simulink model "ATOM_parking_chain"  (R2026a)
settings: Solver=ode4  StopTime=100  FixedStep=0.01
StopFcn:
  | % Put every new figure in the same MATLAB Figures window as a docked tab.
  | set(groot, 'defaultFigureWindowStyle', 'docked');
  | 
  | if exist('costmap_active', 'var') && ...
  |         exist('vehicle', 'var') && ...
  |         exist('parking_path', 'var') && ...
  |         ~isempty(parking_path)
  | 
  |     plotPlan(costmap_active, vehicle, parking_path);
  | 
  | else
  | 
  |     warning('No valid parking path is available for plotting.');
  | 
  | end
  | 
  | PlotControllerReferences( ...
  |     out.controller_reference_log);
  | 
  | PlotControllerTracking( ...
  |     out.controller_tracking_log);
undefined symbols (not defined in the file): lateral, longitudinal, stanley, vehicle
(part 1 of 11)
settings Model: Creator=husain5  LastModifiedBy=husain5
settings HardwareCC: ProdBitPerLong=64.0  ProdHWDeviceType=Intel->x86-64 (Linux 64)

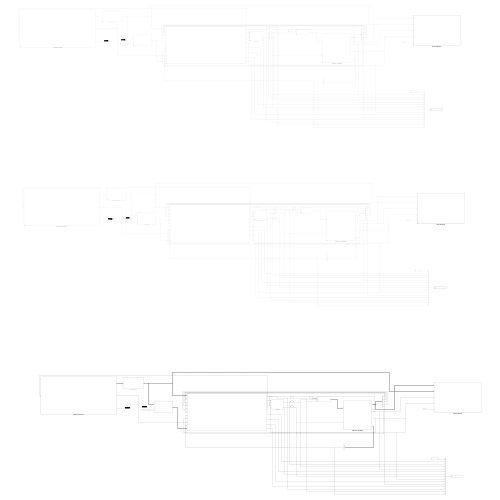
[thumbnail: Simulink's stored preview of the top-level diagram]
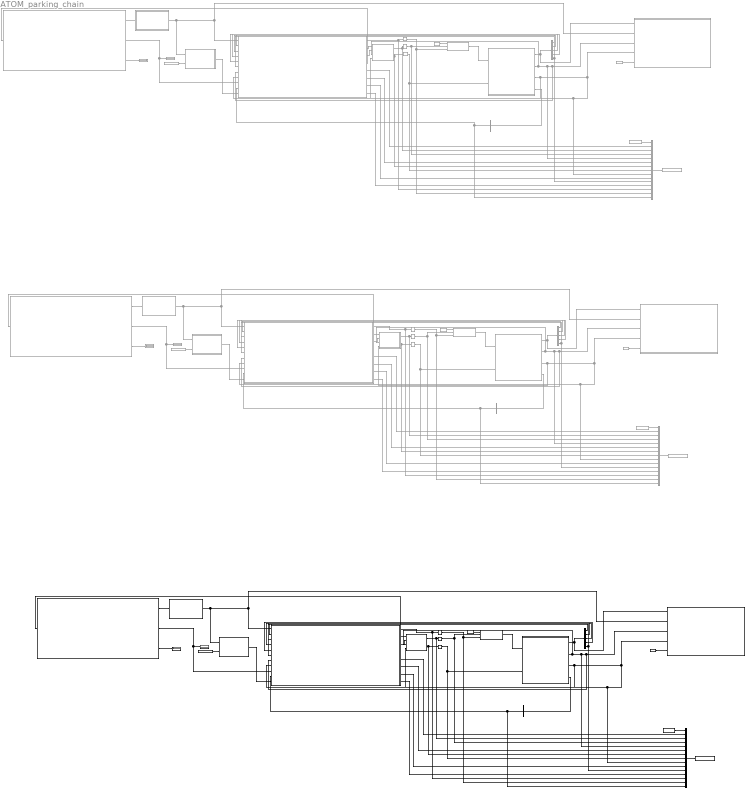
== system ATOM_parking_chain ==
  Bus Assignment : BusAssignment  Commented=on  AssignedSignals=lateral.steering_tire_angle,longitudinal.acceleration
  Bus Assignment1 : BusAssignment  Commented=on  AssignedSignals=lateral.steering_tire_angle,longitudinal.acceleration
  Bus Assignment2 : BusAssignment  AssignedSignals=lateral.steering_tire_angle,longitudinal.acceleration
  Bus Selector1 : BusSelector  Commented=on  OutputSignals=pose.position.x,pose.position.y,pose.orientation.z,pose.orientation.w,twist.linear.x
  Bus Selector2 : BusSelector  Commented=on  OutputSignals=pose.position.x,pose.position.y,pose.orientation.z,pose.orientation.w,twist.linear.x
  Bus Selector3 : BusSelector  Commented=on  OutputSignals=acceleration.linear.x
  Bus Selector4 : BusSelector  Commented=on  OutputSignals=acceleration.linear.x
  Bus Selector5 : BusSelector  OutputSignals=pose.position.x,pose.position.y,pose.orientation.z,pose.orientation.w,twist.linear.x
  Bus Selector6 : BusSelector  OutputSignals=acceleration.linear.x
  Constant : Constant  Commented=on  Value=0  OutDataTypeStr=Bus: ControlCMDBus
  Constant1 : Constant  Commented=on  Value=vehicle.sim.steer_rate_lim
  Constant2 : Constant  Commented=on  Value=0  OutDataTypeStr=Bus: ControlCMDBus
  Constant3 : Constant  Commented=on  Value=vehicle.sim.steer_rate_lim
  Constant4 : Constant  Value=0  OutDataTypeStr=Bus: ControlCMDBus
  Constant5 : Constant  Value=vehicle.sim.steer_rate_lim
  Digital Clock : DigitalClock  Commented=on  SampleTime=0.04
  Digital Clock1 : DigitalClock  Commented=on  SampleTime=0.04
  Digital Clock2 : DigitalClock  SampleTime=0.04
  Display{,1..3} (4 alike) : Display  Commented=on
  Display4 : Display
  Display5 : Display
  From Workspace1 : FromWorkspace  Commented=on  VariableName=veh
  From Workspace2 : FromWorkspace  Commented=on  VariableName=veh
  From Workspace3 : FromWorkspace  VariableName=veh
  Mux1 : Mux  Commented=on  Inputs=15
  Mux2 : Mux  Commented=on  Inputs=15
  Mux3 : Mux  Inputs=15
  Parking Scenario : Subsystem  Commented=on
  Parking Scenario1 : Subsystem  Commented=on
  Parking Scenario2 : Subsystem
  Plot vehicle1 : Subsystem  Commented=on
  Plot vehicle2 : Subsystem  Commented=on
  Plot vehicle3 : Subsystem
  Subsystem : Subsystem  Commented=on
  Subsystem1 : Subsystem  Commented=on
  Subsystem2 : Subsystem
  To Workspace1 : ToWorkspace  Commented=on  VariableName=controller_tracking_log  SaveFormat=Timeseries  SampleTime=-1
  To Workspace2 : ToWorkspace  Commented=on  VariableName=controller_tracking_log2  SaveFormat=Timeseries  SampleTime=-1
  To Workspace3 : ToWorkspace  VariableName=controller_tracking_log  SaveFormat=Timeseries  SampleTime=-1
  Transport Delay : TransportDelay  Commented=on  DelayTime=vehicle.sim.acc_time_delay
  Transport Delay{1..2,4..5} (4 alike) : TransportDelay  Commented=on  DelayTime=vehicle.sim.steer_time_delay
  Transport Delay3 : TransportDelay  Commented=on  DelayTime=vehicle.sim.acc_time_delay
  Transport Delay6 : TransportDelay  DelayTime=vehicle.sim.acc_time_delay
  Transport Delay7 : TransportDelay  DelayTime=vehicle.sim.steer_time_delay
  Transport Delay8 : TransportDelay  DelayTime=vehicle.sim.steer_time_delay
  Vehicle_Model : Subsystem  Commented=on
  Vehicle_Model1 : Subsystem  Commented=on
  Vehicle_Model2 : Subsystem
  parking_velocity_smoother : Subsystem  Commented=on
  parking_velocity_smoother1 : Subsystem  Commented=on
  parking_velocity_smoother2 : Subsystem
  steeringRatetoAngle : Subsystem  Commented=on
  steeringRatetoAngle1 : Subsystem  Commented=on
  steeringRatetoAngle2 : Subsystem
  time_parameterization : Subsystem  Commented=on
  time_parameterization1 : Subsystem  Commented=on
  time_parameterization2 : Subsystem
  wires:
  From Workspace2/1 -> Plot vehicle1/5(veh)
  Constant/1 -> Bus Assignment/1
  Subsystem/4(segment_done) -> Parking Scenario/1(segment_done)
  Subsystem/5(df_ref_out) -> Mux1/2
  Subsystem/1("a_cmd ") -> Transport Delay/1, Mux1/13
  Parking Scenario/1(traj) -> parking_velocity_smoother/1(trajectory_in)
  Bus Selector2/3 -> Subsystem/4(qz)  "<z>"
  Bus Selector2/5 -> Mux1/11, Subsystem/6(vx)  "<x>"
  Bus Selector2/1 -> Subsystem/2(X)  "<x>"
  parking_velocity_smoother/1(trajectory_out) -> time_parameterization/1(trajectory_in), Subsystem/1(planning/scenario_planning/scenario_selector/trajectory), Plot vehicle1/2(planning/scenario_planning/scenario_selector/trajectory)
  Mux1/1 -> To Workspace1/1
  Bus Selector2/4 -> Subsystem/5(qw)  "<w>"
  Subsystem/7(v_ref_out) -> Mux1/10
  Transport Delay1/1 -> Mux1/4, Bus Assignment/2
  Vehicle_Model/3(steer_rear) -> steeringRatetoAngle/4(dr_measured), Mux1/9, Subsystem/8(dr), Plot vehicle1/4(steer_rear)
  Digital Clock/1 -> Mux1/1
  Bus Assignment/1 -> Vehicle_Model/1(command)
  Transport Delay/1 -> Mux1/14, Bus Assignment/3
  Parking Scenario/2(active_segment) -> Subsystem/9(active_segment), Display/1
  Vehicle_Model/1(kinematic) -> Plot vehicle1/1(localization/kinematic_state), Bus Selector2/1  "/localization/kinematic_state"
  Bus Selector3/1 -> Mux1/15, Subsystem/10(ax_meas)  "<x>"
  Transport Delay2/1 -> Mux1/8, Vehicle_Model/2(rear_steer_commanf)
  Bus Selector2/2 -> Subsystem/3(Y)  "<y>"
  Vehicle_Model/2(steer_front) -> steeringRatetoAngle/3(df_measured), Mux1/5, Subsystem/7(df), Plot vehicle1/3(steer_front)
  Parking Scenario/3(maneuver_complete) -> Display1/1
  Subsystem/6(dr_ref_out) -> Mux1/6
  Subsystem/8(a_ref_out) -> Mux1/12
  Vehicle_Model/4(accel) -> Bus Selector3/1  "/localization/acceleration"
  time_parameterization/1(reference_out) -> Subsystem/11(reference_out)
  Constant1/1 -> time_parameterization/2(steer_rate_limit)
  steeringRatetoAngle/2(dr_angle_cmd) -> Transport Delay2/1, Mux1/7
  steeringRatetoAngle/1(df_angle_cmd) -> Transport Delay1/1, Mux1/3
  Subsystem/2(df_cmd) -> steeringRatetoAngle/1(df_rate_cmd)
  Subsystem/3(dr_cmd) -> steeringRatetoAngle/2(dr_rate_cmd)
  Vehicle_Model1/4(accel) -> Bus Selector4/1  "/localization/acceleration"
  Vehicle_Model1/3(steer_rear) -> steeringRatetoAngle1/4(dr_measured), Mux2/9, Subsystem1/8(dr), Plot vehicle2/4(steer_rear)
  Subsystem1/1("a_cmd ") -> Transport Delay3/1, Mux2/13
  Bus Selector1/5 -> Mux2/11, Subsystem1/6(vx)  "<x>"
  Transport Delay4/1 -> Bus Assignment1/2, Mux2/4
  Bus Selector4/1 -> Subsystem1/10(ax_meas), Mux2/15  "<x>"
  Transport Delay5/1 -> Vehicle_Model1/2(rear_steer_commanf), Mux2/8
  Mux2/1 -> To Workspace2/1
  Constant2/1 -> Bus Assignment1/1
  parking_velocity_smoother1/1(trajectory_out) -> time_parameterization1/1(trajectory_in), Subsystem1/1(planning/scenario_planning/scenario_selector/trajectory), Plot vehicle2/2(planning/scenario_planning/scenario_selector/trajectory)
  Subsystem1/6(dr_ref_out) -> Mux2/6
  Parking Scenario1/2(active_segment) -> Subsystem1/9(active_segment), Display2/1
  Subsystem1/5(df_ref_out) -> Mux2/2
  Subsystem1/2(df_cmd) -> steeringRatetoAngle1/1(df_rate_cmd)
  Subsystem1/8(a_ref_out) -> Mux2/12
  time_parameterization1/1(reference_out) -> Subsystem1/11(reference_out)
  Transport Delay3/1 -> Mux2/14, Bus Assignment1/3
  Parking Scenario1/1(traj) -> parking_velocity_smoother1/1(trajectory_in)
  Bus Selector1/2 -> Subsystem1/3(Y)  "<y>"
  Vehicle_Model1/2(steer_front) -> steeringRatetoAngle1/3(df_measured), Mux2/5, Subsystem1/7(df), Plot vehicle2/3(steer_front)
  Constant3/1 -> time_parameterization1/2(steer_rate_limit)
  From Workspace1/1 -> Plot vehicle2/5(veh)
  steeringRatetoAngle1/2(dr_angle_cmd) -> Transport Delay5/1, Mux2/7
  Subsystem1/7(v_ref_out) -> Mux2/10
  Digital Clock1/1 -> Mux2/1
  Subsystem1/3(dr_cmd) -> steeringRatetoAngle1/2(dr_rate_cmd)
  Bus Assignment1/1 -> Vehicle_Model1/1(command)
  Parking Scenario1/3(maneuver_complete) -> Display3/1
  Vehicle_Model1/1(kinematic) -> Plot vehicle2/1(localization/kinematic_state), Bus Selector1/1  "/localization/kinematic_state"
  steeringRatetoAngle1/1(df_angle_cmd) -> Mux2/3, Transport Delay4/1
  Bus Selector1/3 -> Subsystem1/4(qz)  "<z>"
  Bus Selector1/4 -> Subsystem1/5(qw)  "<w>"
  Bus Selector1/1 -> Subsystem1/2(X)  "<x>"
  Subsystem1/4(segment_done) -> Parking Scenario1/1(segment_done)
  Bus Selector5/3 -> Subsystem2/4(qz)  "<z>"
  Parking Scenario2/3(maneuver_complete) -> Display5/1
  parking_velocity_smoother2/1(trajectory_out) -> time_parameterization2/1(trajectory_in), Subsystem2/1(planning/scenario_planning/scenario_selector/trajectory), Plot vehicle3/2(planning/scenario_planning/scenario_selector/trajectory)
  Bus Selector5/2 -> Subsystem2/3(Y)  "<y>"
  Subsystem2/1("a_cmd ") -> Transport Delay6/1, Mux3/13
  Bus Selector6/1 -> Subsystem2/10(ax_meas), Mux3/15  "<x>"
  Vehicle_Model2/4(accel) -> Bus Selector6/1  "/localization/acceleration"
  Subsystem2/8(a_ref_out) -> Mux3/12
  Vehicle_Model2/2(steer_front) -> steeringRatetoAngle2/3(df_measured), Mux3/5, Subsystem2/7(df), Plot vehicle3/3(steer_front)
  Subsystem2/6(dr_ref_out) -> Mux3/6
  Bus Selector5/1 -> Subsystem2/2(X)  "<x>"
  time_parameterization2/1(reference_out) -> Subsystem2/11(reference_out)
  Subsystem2/7(v_ref_out) -> Mux3/10
  Constant5/1 -> time_parameterization2/2(steer_rate_limit)
  Vehicle_Model2/3(steer_rear) -> steeringRatetoAngle2/4(dr_measured), Mux3/9, Subsystem2/8(dr), Plot vehicle3/4(steer_rear)
  Subsystem2/4(segment_done) -> Parking Scenario2/1(segment_done)
  Constant4/1 -> Bus Assignment2/1
  steeringRatetoAngle2/2(dr_angle_cmd) -> Transport Delay8/1, Mux3/7
  Subsystem2/2(df_cmd) -> steeringRatetoAngle2/1(df_rate_cmd)
  Digital Clock2/1 -> Mux3/1
  Transport Delay6/1 -> Mux3/14, Bus Assignment2/3
  Mux3/1 -> To Workspace3/1
  Parking Scenario2/1(traj) -> parking_velocity_smoother2/1(trajectory_in)
  Bus Selector5/4 -> Subsystem2/5(qw)  "<w>"
  Subsystem2/5(df_ref_out) -> Mux3/2
  Bus Selector5/5 -> Mux3/11, Subsystem2/6(vx)  "<x>"
  steeringRatetoAngle2/1(df_angle_cmd) -> Mux3/3, Transport Delay7/1
  Transport Delay7/1 -> Bus Assignment2/2, Mux3/4
  Transport Delay8/1 -> Vehicle_Model2/2(rear_steer_commanf), Mux3/8
  Vehicle_Model2/1(kinematic) -> Plot vehicle3/1(localization/kinematic_state), Bus Selector5/1  "/localization/kinematic_state"
  Bus Assignment2/1 -> Vehicle_Model2/1(command)
  Parking Scenario2/2(active_segment) -> Subsystem2/9(active_segment), Display4/1
  From Workspace3/1 -> Plot vehicle3/5(veh)
  Subsystem2/3(dr_cmd) -> steeringRatetoAngle2/2(dr_rate_cmd)

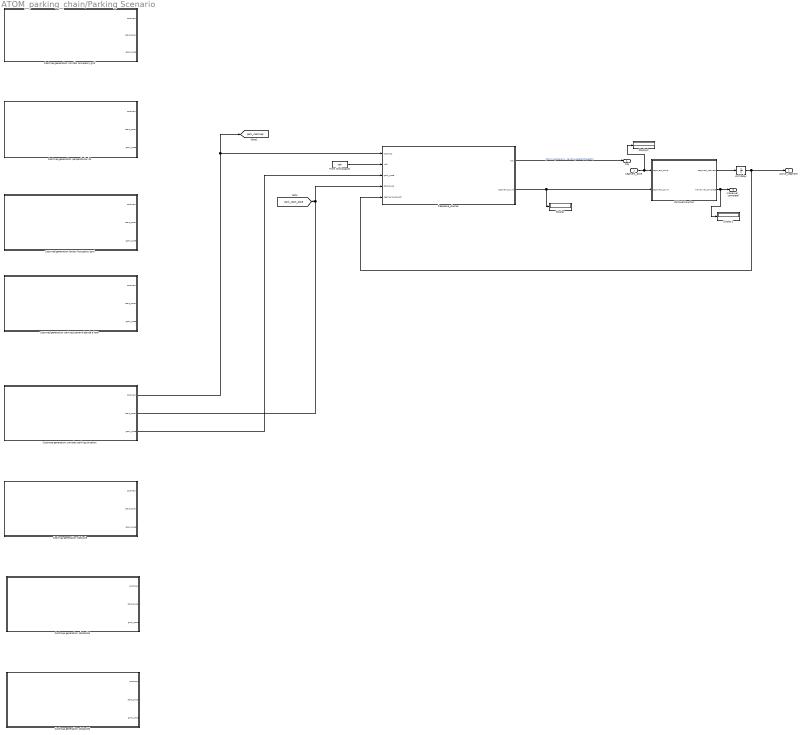
== system ATOM_parking_chain/Parking Scenario ==
  segment_done : Inport
  Costmap generation: complex parking situation : Subsystem
  Costmap generation: corridor occupancy grid : Subsystem
  Costmap generation: empty occupancy grid : Subsystem
  Costmap generation: obstacle : Subsystem
  Costmap generation: obstacle1 : Subsystem
  Costmap generation: obstacle2 : Subsystem
  Costmap generation: parking scenario beside a lane : Subsystem
  Costmap generation: perpendicular lot : Subsystem
  Display : Display
  Display1 : Display
  Display2 : Display
  From Workspace1 : FromWorkspace  VariableName=veh
  MATLAB Function : MATLAB Function  TreatAsAtomicUnit=on
  Unit Delay : UnitDelay  InitialCondition=1  SampleTime=0.04
  freespace_planner : Subsystem
  traj : Outport
  active_segment : Outport  Port=2
  maneuver_complete : Outport  Port=3
  tag scope: park_costmap=global, park_start_pose=global
  wires:
  Costmap generation: complex parking situation/1(costmap) -> [park_costmap], freespace_planner/1(costmap)
  From Workspace1/1 -> freespace_planner/2(veh)
  Costmap generation: complex parking situation/3(goal_pose) -> freespace_planner/3(goal_pose)
  Costmap generation: complex parking situation/2(start_pose) -> freespace_planner/4(start_pose), [park_start_pose]
  freespace_planner/1(traj) -> traj/1  "/planning/scenario_planning/scenario_selector/trajectory"
  Unit Delay/1 -> freespace_planner/5(segment_request), active_segment/1
  freespace_planner/2(segment_count) -> Display/1, MATLAB Function/2(segment_count)
  segment_done/1 -> Display2/1, MATLAB Function/1(segment_done)
  MATLAB Function/1(segment_request) -> Unit Delay/1
  MATLAB Function/2(maneuver_complete) -> Display1/1, maneuver_complete/1

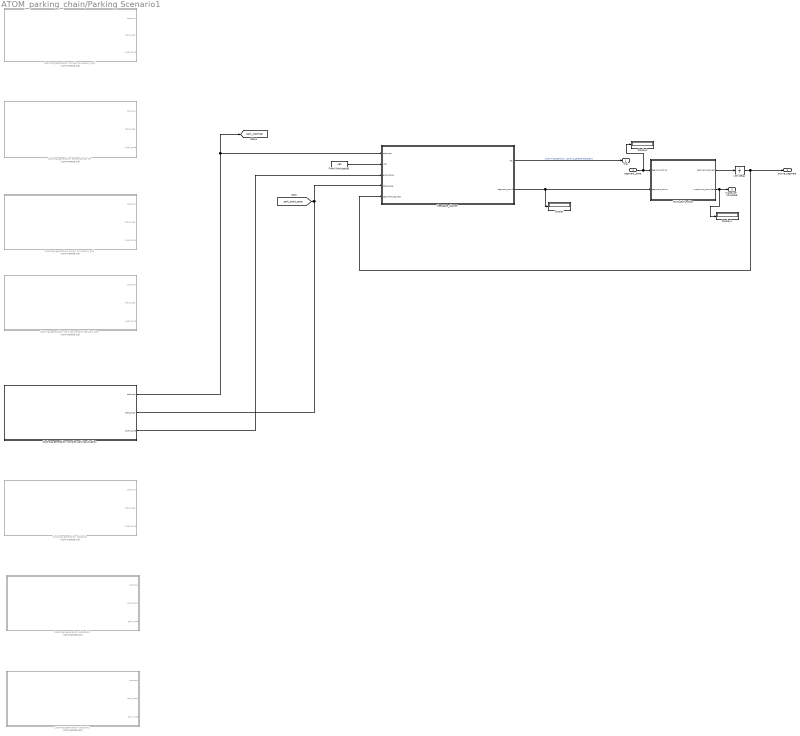
== system ATOM_parking_chain/Parking Scenario1 ==
  segment_done : Inport
  Costmap generation: complex parking situation : Subsystem
  Costmap generation: corridor occupancy grid : Subsystem  Commented=on
  Costmap generation: empty occupancy grid : Subsystem  Commented=on
  Costmap generation: obstacle : Subsystem  Commented=on
  Costmap generation: obstacle1 : Subsystem  Commented=on
  Costmap generation: obstacle2 : Subsystem  Commented=on
  Costmap generation: parking scenario beside a lane : Subsystem  Commented=on
  Costmap generation: perpendicular lot : Subsystem  Commented=on
  Display : Display
  Display1 : Display
  Display2 : Display
  From Workspace1 : FromWorkspace  VariableName=veh
  MATLAB Function : MATLAB Function  TreatAsAtomicUnit=on
  Unit Delay : UnitDelay  InitialCondition=1  SampleTime=0.04
  freespace_planner : Subsystem
  traj : Outport
  active_segment : Outport  Port=2
  maneuver_complete : Outport  Port=3
  tag scope: park_costmap=global, park_start_pose=global
  wires:
  Costmap generation: complex parking situation/1(costmap) -> [park_costmap], freespace_planner/1(costmap)
  From Workspace1/1 -> freespace_planner/2(veh)
  Costmap generation: complex parking situation/3(goal_pose) -> freespace_planner/3(goal_pose)
  Costmap generation: complex parking situation/2(start_pose) -> freespace_planner/4(start_pose), [park_start_pose]
  freespace_planner/1(traj) -> traj/1  "/planning/scenario_planning/scenario_selector/trajectory"
  Unit Delay/1 -> freespace_planner/5(segment_request), active_segment/1
  freespace_planner/2(segment_count) -> Display/1, MATLAB Function/2(segment_count)
  segment_done/1 -> Display2/1, MATLAB Function/1(segment_done)
  MATLAB Function/1(segment_request) -> Unit Delay/1
  MATLAB Function/2(maneuver_complete) -> Display1/1, maneuver_complete/1

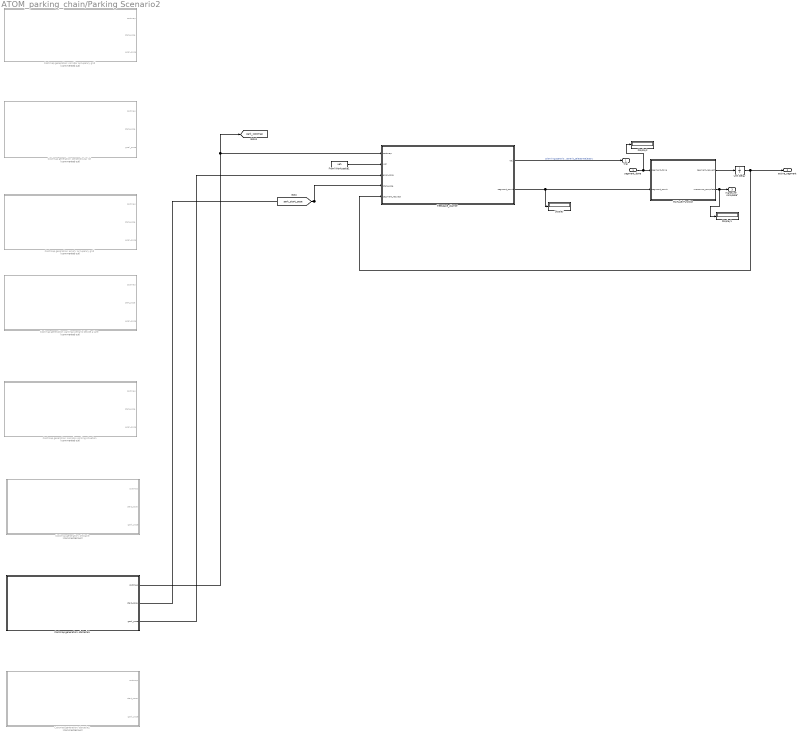
== system ATOM_parking_chain/Parking Scenario2 ==
  segment_done : Inport
  Costmap generation: complex parking situation : Subsystem  Commented=on
  Costmap generation: corridor occupancy grid : Subsystem  Commented=on
  Costmap generation: empty occupancy grid : Subsystem  Commented=on
  Costmap generation: obstacle : Subsystem  Commented=on
  Costmap generation: obstacle1 : Subsystem
  Costmap generation: obstacle2 : Subsystem  Commented=on
  Costmap generation: parking scenario beside a lane : Subsystem  Commented=on
  Costmap generation: perpendicular lot : Subsystem  Commented=on
  Display : Display
  Display1 : Display
  Display2 : Display
  From Workspace1 : FromWorkspace  VariableName=veh
  MATLAB Function : MATLAB Function  TreatAsAtomicUnit=on
  Unit Delay : UnitDelay  InitialCondition=1  SampleTime=0.04
  freespace_planner : Subsystem
  traj : Outport
  active_segment : Outport  Port=2
  maneuver_complete : Outport  Port=3
  tag scope: park_costmap=global, park_start_pose=global
  wires:
  Costmap generation: obstacle1/1(costmap) -> [park_costmap], freespace_planner/1(costmap)
  From Workspace1/1 -> freespace_planner/2(veh)
  Costmap generation: obstacle1/3(goal_pose) -> freespace_planner/3(goal_pose)
  Costmap generation: obstacle1/2(start_pose) -> freespace_planner/4(start_pose), [park_start_pose]
  freespace_planner/1(traj) -> traj/1  "/planning/scenario_planning/scenario_selector/trajectory"
  Unit Delay/1 -> freespace_planner/5(segment_request), active_segment/1
  freespace_planner/2(segment_count) -> Display/1, MATLAB Function/2(segment_count)
  segment_done/1 -> Display2/1, MATLAB Function/1(segment_done)
  MATLAB Function/1(segment_request) -> Unit Delay/1
  MATLAB Function/2(maneuver_complete) -> Display1/1, maneuver_complete/1

== system ATOM_parking_chain/Plot vehicle1 ==
  localization/kinematic_state : Inport
  planning/scenario_planning/scenario_selector/trajectory : Inport  Port=2
  steer_front : Inport  Port=3
  steer_rear : Inport  Port=4
  veh : Inport  Port=5
  Constant : Constant  Value=vehicle.param.wheel_base
  Plot Vehicle Rear reference frame : MATLAB Function  TreatAsAtomicUnit=on
  Plot vehicle Front reference frame : MATLAB Function  TreatAsAtomicUnit=on
  RearToFrontOdometry : MATLAB Function  TreatAsAtomicUnit=on
  SetStanleyTrajectory : Subsystem
  wires:
  steer_rear/1 -> Plot vehicle Front reference frame/3(steer_rear), Plot Vehicle Rear reference frame/3(steer_rear)
  veh/1 -> Plot vehicle Front reference frame/4(veh), Plot Vehicle Rear reference frame/4(veh)
  steer_front/1 -> Plot Vehicle Rear reference frame/2(steer_front), Plot vehicle Front reference frame/2(steer_front)
  Constant/1 -> RearToFrontOdometry/2(wheel_base)
  localization/kinematic_state/1 -> Plot Vehicle Rear reference frame/1(kinematic), RearToFrontOdometry/1(rear_pose)
  planning/scenario_planning/scenario_selector/trajectory/1 -> SetStanleyTrajectory/1(ref_traj), Plot Vehicle Rear reference frame/5(traj)
  RearToFrontOdometry/1(front_pose) -> SetStanleyTrajectory/2(ego_pose), Plot vehicle Front reference frame/1(kinematic)
  SetStanleyTrajectory/1(trajectory_out) -> Plot vehicle Front reference frame/5(traj)
  [park_costmap] -> Plot Vehicle Rear reference frame/6(costmap)

== system ATOM_parking_chain/Plot vehicle2 ==
  localization/kinematic_state : Inport
  planning/scenario_planning/scenario_selector/trajectory : Inport  Port=2
  steer_front : Inport  Port=3
  steer_rear : Inport  Port=4
  veh : Inport  Port=5
  Constant : Constant  Value=vehicle.param.wheel_base
  Plot Vehicle Rear reference frame : MATLAB Function  TreatAsAtomicUnit=on
  Plot vehicle Front reference frame : MATLAB Function  TreatAsAtomicUnit=on
  RearToFrontOdometry : MATLAB Function  TreatAsAtomicUnit=on
  SetStanleyTrajectory : Subsystem
  wires:
  steer_rear/1 -> Plot vehicle Front reference frame/3(steer_rear), Plot Vehicle Rear reference frame/3(steer_rear)
  veh/1 -> Plot vehicle Front reference frame/4(veh), Plot Vehicle Rear reference frame/4(veh)
  steer_front/1 -> Plot Vehicle Rear reference frame/2(steer_front), Plot vehicle Front reference frame/2(steer_front)
  Constant/1 -> RearToFrontOdometry/2(wheel_base)
  localization/kinematic_state/1 -> Plot Vehicle Rear reference frame/1(kinematic), RearToFrontOdometry/1(rear_pose)
  planning/scenario_planning/scenario_selector/trajectory/1 -> SetStanleyTrajectory/1(ref_traj), Plot Vehicle Rear reference frame/5(traj)
  RearToFrontOdometry/1(front_pose) -> SetStanleyTrajectory/2(ego_pose), Plot vehicle Front reference frame/1(kinematic)
  SetStanleyTrajectory/1(trajectory_out) -> Plot vehicle Front reference frame/5(traj)
  [park_costmap] -> Plot Vehicle Rear reference frame/6(costmap)

== system ATOM_parking_chain/Plot vehicle3 ==
  localization/kinematic_state : Inport
  planning/scenario_planning/scenario_selector/trajectory : Inport  Port=2
  steer_front : Inport  Port=3
  steer_rear : Inport  Port=4
  veh : Inport  Port=5
  Constant : Constant  Value=vehicle.param.wheel_base
  Plot Vehicle Rear reference frame : MATLAB Function  TreatAsAtomicUnit=on
  Plot vehicle Front reference frame : MATLAB Function  TreatAsAtomicUnit=on
  RearToFrontOdometry : MATLAB Function  TreatAsAtomicUnit=on
  SetStanleyTrajectory : Subsystem
  wires:
  steer_rear/1 -> Plot vehicle Front reference frame/3(steer_rear), Plot Vehicle Rear reference frame/3(steer_rear)
  veh/1 -> Plot vehicle Front reference frame/4(veh), Plot Vehicle Rear reference frame/4(veh)
  steer_front/1 -> Plot Vehicle Rear reference frame/2(steer_front), Plot vehicle Front reference frame/2(steer_front)
  Constant/1 -> RearToFrontOdometry/2(wheel_base)
  localization/kinematic_state/1 -> Plot Vehicle Rear reference frame/1(kinematic), RearToFrontOdometry/1(rear_pose)
  planning/scenario_planning/scenario_selector/trajectory/1 -> SetStanleyTrajectory/1(ref_traj), Plot Vehicle Rear reference frame/5(traj)
  RearToFrontOdometry/1(front_pose) -> SetStanleyTrajectory/2(ego_pose), Plot vehicle Front reference frame/1(kinematic)
  SetStanleyTrajectory/1(trajectory_out) -> Plot vehicle Front reference frame/5(traj)
  [park_costmap] -> Plot Vehicle Rear reference frame/6(costmap)

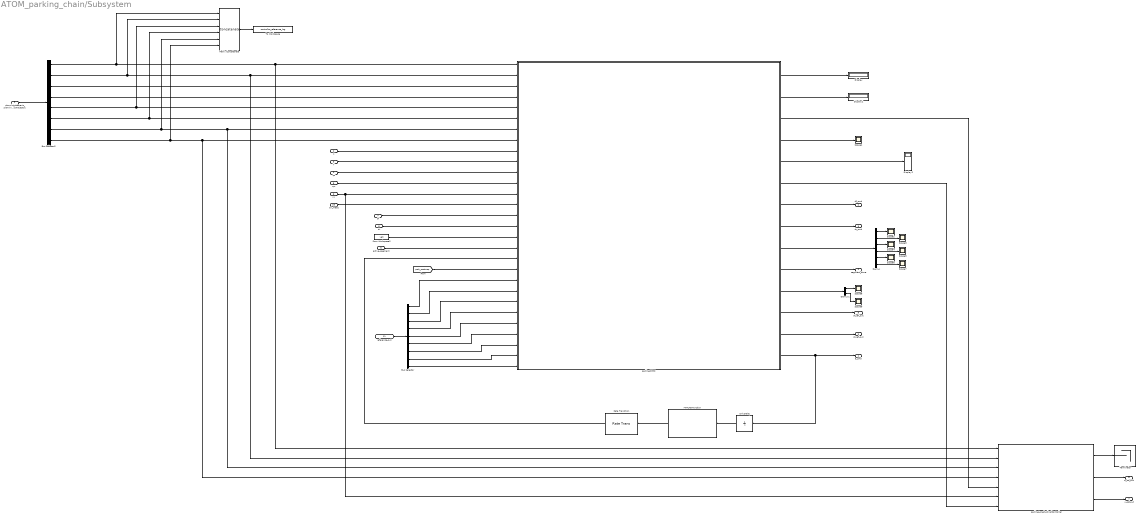
== system ATOM_parking_chain/Subsystem ==
  planning/scenario_planning/scenario_selector/trajectory : Inport
  X : Inport  Port=2
  Y : Inport  Port=3
  qz : Inport  Port=4
  qw : Inport  Port=5
  vx : Inport  Port=6
  df : Inport  Port=7
  dr : Inport  Port=8
  active_segment : Inport  Port=9
  ax_meas : Inport  Port=10
  reference_out : Inport  Port=11  OutDataTypeStr=Bus: ParkingReferenceBus  PortDimensions=1
  Bus Selector : BusSelector  OutputSignals=t_ref,s_ref,x_ref,y_ref,psi_ref,v_ref,a_ref,df_nom,dr_nom
  Bus Selector2 : BusSelector  OutputSignals=pose.position.x,pose.position.y,pose.orientation.qz,pose.orientation.qw,front_wheel_angle_rad,rear_wheel_angle_rad,longitudinal_velocity_mps,acceleration_mps2
  Demux : Demux  Outputs=6
  Demux1 : Demux  Outputs=2
  Display : Display
  Display1 : Display
  Display2 : Display
  From Workspace2 : FromWorkspace  VariableName=veh
  MATLAB Function : MATLAB Function  TreatAsAtomicUnit=on
  Matrix Concatenate : Concatenate  NumInputs=6  Mode=Multidimensional array  ConcatenateDimension=2
  Rate Transition : RateTransition  OutPortSampleTime=0.04
  Scope{1..9} (9 alike) : Scope
      Scope1 settings: ActiveDisplayYMinimum=-1  ActiveDisplayYMaximum=1  DataLoggingVariableName=ScopeData8
      Scope2 settings: ActiveDisplayYMinimum=-10.60989505612366  ActiveDisplayYMaximum=95.489308452219746  DataLoggingVariableName=ScopeData7
      Scope3 settings: ActiveDisplayYMinimum=-0.24999999999999994  ActiveDisplayYMaximum=2.25  DataLoggingVariableName=ScopeData8
      Scope4 settings: ActiveDisplayYMinimum=-0.028305171249999993  ActiveDisplayYMaximum=0.28435258124999996  DataLoggingVariableName=ScopeData9
      Scope5 settings: ActiveDisplayYMinimum=-3.7094155844155834  ActiveDisplayYMaximum=33.790584415584412  DataLoggingVariableName=ScopeData10
      Scope6 settings: ActiveDisplayYMinimum=-91.999999999999972  ActiveDisplayYMaximum=1138  DataLoggingVariableName=ScopeData11
      Scope7 settings: ActiveDisplayYMinimum=-0.87499999999999978  ActiveDisplayYMaximum=7.875  DataLoggingVariableName=ScopeData12
      Scope8 settings: ActiveDisplayYMinimum=-1.2636206575927895  ActiveDisplayYMaximum=11.514759920051633  DataLoggingVariableName=ScopeData13
      Scope9 settings: ActiveDisplayYMinimum=-11.039926031619149  ActiveDisplayYMaximum=66.9081819483468  DataLoggingVariableName=ScopeData14
  Terminator : Terminator
  To Workspace : ToWorkspace  VariableName=controller_reference_log  SampleTime=-1
  Unit Delay : UnitDelay  SampleTime=0.04
  parkingLongitudinalController : MATLAB Function  TreatAsAtomicUnit=on
  parkingNMPC : MATLAB Function  TreatAsAtomicUnit=on
  "a_cmd " : Outport
  df_cmd : Outport  Port=2
  dr_cmd : Outport  Port=3
  segment_done : Outport  Port=4
  df_ref_out : Outport  Port=5
  dr_ref_out : Outport  Port=6
  v_ref_out : Outport  Port=7
  a_ref_out : Outport  Port=8
  wires:
  Bus Selector2/5 -> Matrix Concatenate/3, parkingNMPC/5(tdf)  "<front_wheel_angle_rad>"
  parkingNMPC/2(max_q) -> Display1/1
  Bus Selector2/2 -> Matrix Concatenate/2, parkingLongitudinalController/2(ty), parkingNMPC/2(ty)  "<y>"
  Bus Selector2/4 -> parkingNMPC/4(tqw)  "<qw>"
  Bus Selector2/3 -> parkingNMPC/3(tqz)  "<qz>"
  Bus Selector2/1 -> parkingNMPC/1(tx), parkingLongitudinalController/1(tx), Matrix Concatenate/1  "<x>"
  parkingNMPC/1(path_length) -> Display/1
  Bus Selector2/6 -> Matrix Concatenate/4, parkingNMPC/6(tdr)  "<rear_wheel_angle_rad>"
  planning/scenario_planning/scenario_selector/trajectory/1 -> Bus Selector2/1
  X/1 -> parkingNMPC/9(X)
  Y/1 -> parkingNMPC/10(Y)
  parkingNMPC/3(s_now) -> parkingLongitudinalController/5(s_now)
  parkingNMPC/4(ey_now) -> Scope1/1
  qz/1 -> parkingNMPC/11(qz)
  qw/1 -> parkingNMPC/12(qw)
  vx/1 -> parkingNMPC/13(vx), parkingLongitudinalController/6(vx)
  df/1 -> parkingNMPC/15(df)
  dr/1 -> parkingNMPC/16(dr)
  parkingNMPC/5(x_now) -> Display2/1
  From Workspace2/1 -> parkingNMPC/17(veh)
  parkingNMPC/6(longitudinal_mode) -> parkingLongitudinalController/7(longitudinal_mode)
  parkingNMPC/7(df_rate_cmd) -> df_cmd/1
  parkingNMPC/8(dr_rate_cmd) -> dr_cmd/1
  parkingNMPC/9(nmpc_info) -> Demux/1
  Demux/1 -> Scope2/1
  Demux/2 -> Scope3/1
  Demux/3 -> Scope4/1
  Demux/4 -> Scope5/1
  Demux/5 -> Scope6/1
  Demux/6 -> Scope7/1
  Bus Selector2/7 -> Matrix Concatenate/5, parkingNMPC/7(tvx), parkingLongitudinalController/3(tvx)  "<longitudinal_velocity_mps>"
  parkingNMPC/10(segment_done) -> segment_done/1
  active_segment/1 -> parkingNMPC/18(active_segment)
  parkingNMPC/11(endpoint_error) -> Demux1/1
  Demux1/1 -> Scope8/1
  Demux1/2 -> Scope9/1
  Bus Selector2/8 -> Matrix Concatenate/6, parkingLongitudinalController/4(tax), parkingNMPC/8(tax)  "<acceleration_mps2>"
  ax_meas/1 -> parkingNMPC/14(ax_meas)
  MATLAB Function/1(a_cmd_history) -> Rate Transition/1
  parkingLongitudinalController/2(a_ref_out) -> a_ref_out/1
  [park_costmap] -> parkingNMPC/20(costmap)
  Matrix Concatenate/1 -> To Workspace/1
  parkingNMPC/12(df_ref_out) -> df_ref_out/1
  parkingNMPC/13(dr_ref_out) -> dr_ref_out/1
  parkingLongitudinalController/3(v_ref_out) -> v_ref_out/1
  reference_out/1 -> Bus Selector/1
  Bus Selector/1 -> parkingNMPC/21(t_ref)  "<t_ref>"
  Bus Selector/2 -> parkingNMPC/22(s_ref)  "<s_ref>"
  Bus Selector/3 -> parkingNMPC/23(x_ref)  "<x_ref>"
  Bus Selector/4 -> parkingNMPC/24(y_ref)  "<y_ref>"
  Bus Selector/5 -> parkingNMPC/25(psi_ref)  "<psi_ref>"
  Bus Selector/6 -> parkingNMPC/26(v_ref)  "<v_ref>"
  Bus Selector/7 -> parkingNMPC/27(a_ref)  "<a_ref>"
  Bus Selector/8 -> parkingNMPC/28(df_nom)  "<df_nom>"
  Bus Selector/9 -> parkingNMPC/29(dr_nom)  "<dr_nom>"
  Unit Delay/1 -> MATLAB Function/1(a_cmd_previous)
  Rate Transition/1 -> parkingNMPC/19(a_cmd_history)
  parkingNMPC/14(a_cmd_nmpc) -> Unit Delay/1, "a_cmd "/1
  parkingLongitudinalController/1(a_cmd) -> Terminator/1

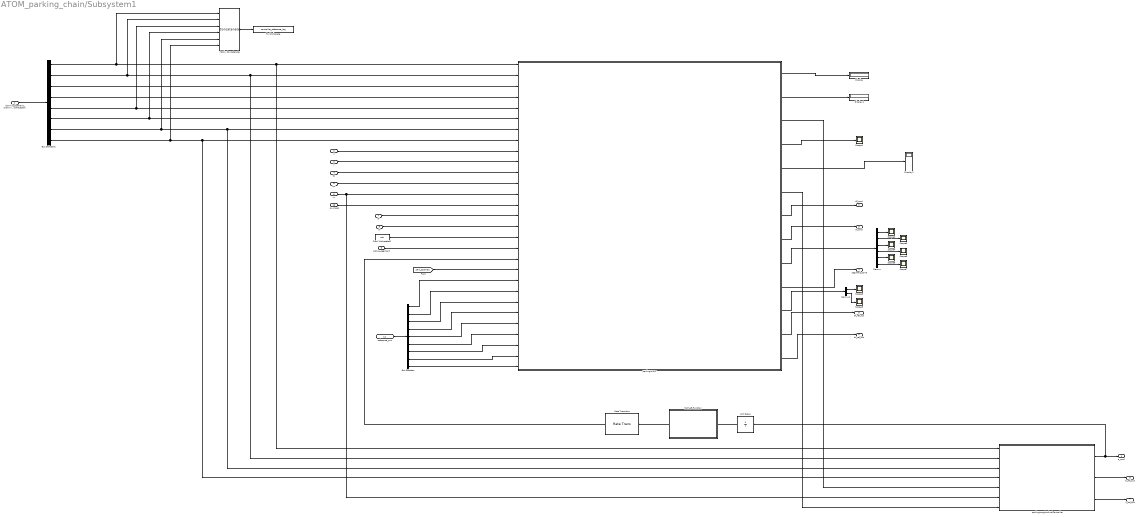
== system ATOM_parking_chain/Subsystem1 ==
  planning/scenario_planning/scenario_selector/trajectory : Inport
  X : Inport  Port=2
  Y : Inport  Port=3
  qz : Inport  Port=4
  qw : Inport  Port=5
  vx : Inport  Port=6
  df : Inport  Port=7
  dr : Inport  Port=8
  active_segment : Inport  Port=9
  ax_meas : Inport  Port=10
  reference_out : Inport  Port=11  OutDataTypeStr=Bus: ParkingReferenceBus  PortDimensions=1
  Bus Selector : BusSelector  OutputSignals=t_ref,s_ref,x_ref,y_ref,psi_ref,v_ref,a_ref,df_nom,dr_nom
  Bus Selector2 : BusSelector  OutputSignals=pose.position.x,pose.position.y,pose.orientation.qz,pose.orientation.qw,front_wheel_angle_rad,rear_wheel_angle_rad,longitudinal_velocity_mps,acceleration_mps2
  Demux : Demux  Outputs=6
  Demux1 : Demux  Outputs=2
  Display : Display
  Display1 : Display
  Display2 : Display
  From Workspace2 : FromWorkspace  VariableName=veh
  MATLAB Function : MATLAB Function  TreatAsAtomicUnit=on
  Matrix Concatenate : Concatenate  NumInputs=6  Mode=Multidimensional array  ConcatenateDimension=2
  Rate Transition : RateTransition  OutPortSampleTime=0.04
  Scope{1..9} (9 alike) : Scope
      Scope1 settings: ActiveDisplayYMinimum=-1  ActiveDisplayYMaximum=1  DataLoggingVariableName=ScopeData8
      Scope2 settings: ActiveDisplayYMinimum=-10.60989505612366  ActiveDisplayYMaximum=95.489308452219746  DataLoggingVariableName=ScopeData7
      Scope3 settings: ActiveDisplayYMinimum=-0.24999999999999994  ActiveDisplayYMaximum=2.25  DataLoggingVariableName=ScopeData8
      Scope4 settings: ActiveDisplayYMinimum=-0.028305171249999993  ActiveDisplayYMaximum=0.28435258124999996  DataLoggingVariableName=ScopeData9
      Scope5 settings: ActiveDisplayYMinimum=-3.7094155844155834  ActiveDisplayYMaximum=33.790584415584412  DataLoggingVariableName=ScopeData10
      Scope6 settings: ActiveDisplayYMinimum=-91.999999999999972  ActiveDisplayYMaximum=1138  DataLoggingVariableName=ScopeData11
      Scope7 settings: ActiveDisplayYMinimum=-0.87499999999999978  ActiveDisplayYMaximum=7.875  DataLoggingVariableName=ScopeData12
      Scope8 settings: ActiveDisplayYMinimum=-1.2636206575927895  ActiveDisplayYMaximum=11.514759920051633  DataLoggingVariableName=ScopeData13
      Scope9 settings: ActiveDisplayYMinimum=-11.039926031619149  ActiveDisplayYMaximum=66.9081819483468  DataLoggingVariableName=ScopeData14
  To Workspace : ToWorkspace  VariableName=controller_reference_log  SampleTime=-1
  Unit Delay : UnitDelay  SampleTime=0.04
  parkingLongitudinalController : MATLAB Function  TreatAsAtomicUnit=on
  parkingNMPC : MATLAB Function  TreatAsAtomicUnit=on
  "a_cmd " : Outport
  df_cmd : Outport  Port=2
  dr_cmd : Outport  Port=3
  segment_done : Outport  Port=4
  df_ref_out : Outport  Port=5
  dr_ref_out : Outport  Port=6
  v_ref_out : Outport  Port=7
  a_ref_out : Outport  Port=8
  wires:
  Bus Selector2/5 -> Matrix Concatenate/3, parkingNMPC/5(tdf)  "<front_wheel_angle_rad>"
  parkingNMPC/2(max_q) -> Display1/1
  Bus Selector2/2 -> Matrix Concatenate/2, parkingLongitudinalController/2(ty), parkingNMPC/2(ty)  "<y>"
  Bus Selector2/4 -> parkingNMPC/4(tqw)  "<qw>"
  Bus Selector2/3 -> parkingNMPC/3(tqz)  "<qz>"
  Bus Selector2/1 -> parkingNMPC/1(tx), parkingLongitudinalController/1(tx), Matrix Concatenate/1  "<x>"
  parkingNMPC/1(path_length) -> Display/1
  Bus Selector2/6 -> Matrix Concatenate/4, parkingNMPC/6(tdr)  "<rear_wheel_angle_rad>"
  planning/scenario_planning/scenario_selector/trajectory/1 -> Bus Selector2/1
  X/1 -> parkingNMPC/9(X)
  Y/1 -> parkingNMPC/10(Y)
  parkingNMPC/3(s_now) -> parkingLongitudinalController/5(s_now)
  parkingNMPC/4(ey_now) -> Scope1/1
  qz/1 -> parkingNMPC/11(qz)
  qw/1 -> parkingNMPC/12(qw)
  vx/1 -> parkingNMPC/13(vx), parkingLongitudinalController/6(vx)
  df/1 -> parkingNMPC/15(df)
  dr/1 -> parkingNMPC/16(dr)
  parkingNMPC/5(x_now) -> Display2/1
  From Workspace2/1 -> parkingNMPC/17(veh)
  parkingNMPC/6(longitudinal_mode) -> parkingLongitudinalController/7(longitudinal_mode)
  parkingNMPC/7(df_rate_cmd) -> df_cmd/1
  parkingNMPC/8(dr_rate_cmd) -> dr_cmd/1
  parkingNMPC/9(nmpc_info) -> Demux/1
  Demux/1 -> Scope2/1
  Demux/2 -> Scope3/1
  Demux/3 -> Scope4/1
  Demux/4 -> Scope5/1
  Demux/5 -> Scope6/1
  Demux/6 -> Scope7/1
  Bus Selector2/7 -> Matrix Concatenate/5, parkingNMPC/7(tvx), parkingLongitudinalController/3(tvx)  "<longitudinal_velocity_mps>"
  parkingNMPC/10(segment_done) -> segment_done/1
  active_segment/1 -> parkingNMPC/18(active_segment)
  parkingNMPC/11(endpoint_error) -> Demux1/1
  Demux1/1 -> Scope8/1
  Demux1/2 -> Scope9/1
  Bus Selector2/8 -> Matrix Concatenate/6, parkingLongitudinalController/4(tax), parkingNMPC/8(tax)  "<acceleration_mps2>"
  ax_meas/1 -> parkingNMPC/14(ax_meas)
  MATLAB Function/1(a_cmd_history) -> Rate Transition/1
  parkingLongitudinalController/2(a_ref_out) -> a_ref_out/1
  [park_costmap] -> parkingNMPC/20(costmap)
  Matrix Concatenate/1 -> To Workspace/1
  parkingNMPC/12(df_ref_out) -> df_ref_out/1
  parkingNMPC/13(dr_ref_out) -> dr_ref_out/1
  parkingLongitudinalController/3(v_ref_out) -> v_ref_out/1
  reference_out/1 -> Bus Selector/1
  Bus Selector/1 -> parkingNMPC/21(t_ref)  "<t_ref>"
  Bus Selector/2 -> parkingNMPC/22(s_ref)  "<s_ref>"
  Bus Selector/3 -> parkingNMPC/23(x_ref)  "<x_ref>"
  Bus Selector/4 -> parkingNMPC/24(y_ref)  "<y_ref>"
  Bus Selector/5 -> parkingNMPC/25(psi_ref)  "<psi_ref>"
  Bus Selector/6 -> parkingNMPC/26(v_ref)  "<v_ref>"
  Bus Selector/7 -> parkingNMPC/27(a_ref)  "<a_ref>"
  Bus Selector/8 -> parkingNMPC/28(df_nom)  "<df_nom>"
  Bus Selector/9 -> parkingNMPC/29(dr_nom)  "<dr_nom>"
  Unit Delay/1 -> MATLAB Function/1(a_cmd_previous)
  Rate Transition/1 -> parkingNMPC/19(a_cmd_history)
  parkingLongitudinalController/1(a_cmd) -> Unit Delay/1, "a_cmd "/1

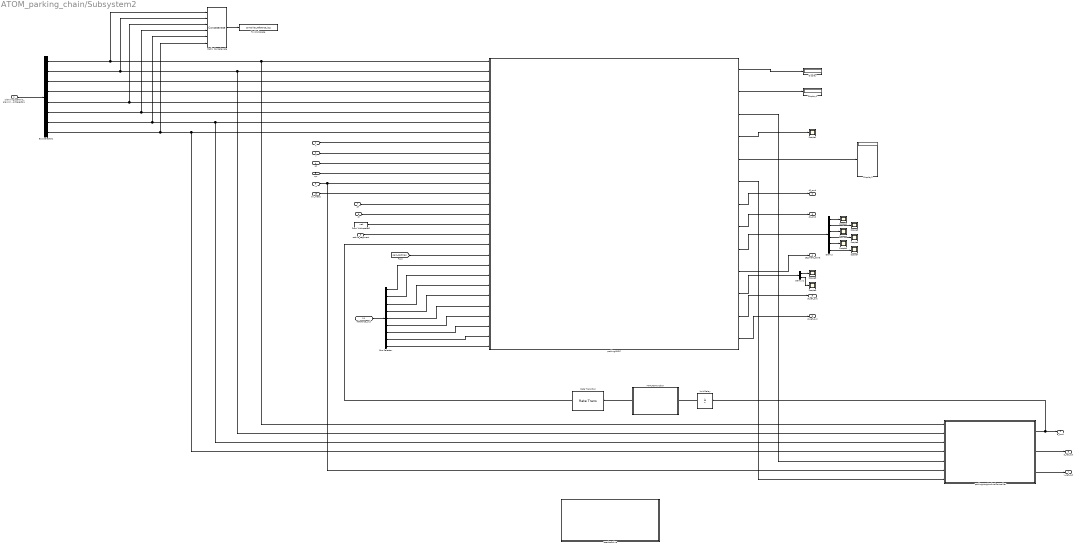
== system ATOM_parking_chain/Subsystem2 ==
  planning/scenario_planning/scenario_selector/trajectory : Inport
  X : Inport  Port=2
  Y : Inport  Port=3
  qz : Inport  Port=4
  qw : Inport  Port=5
  vx : Inport  Port=6
  df : Inport  Port=7
  dr : Inport  Port=8
  active_segment : Inport  Port=9
  ax_meas : Inport  Port=10
  reference_out : Inport  Port=11  OutDataTypeStr=Bus: ParkingReferenceBus  PortDimensions=1
  Bus Selector : BusSelector  OutputSignals=t_ref,s_ref,x_ref,y_ref,psi_ref,v_ref,a_ref,df_nom,dr_nom
  Bus Selector2 : BusSelector  OutputSignals=pose.position.x,pose.position.y,pose.orientation.qz,pose.orientation.qw,front_wheel_angle_rad,rear_wheel_angle_rad,longitudinal_velocity_mps,acceleration_mps2
  Demux : Demux  Outputs=6
  Demux1 : Demux  Outputs=2
  Display : Display
  Display1 : Display
  Display2 : Display
  From Workspace2 : FromWorkspace  VariableName=veh
  MATLAB Function : MATLAB Function  TreatAsAtomicUnit=on
  Matrix Concatenate : Concatenate  NumInputs=6  Mode=Multidimensional array  ConcatenateDimension=2
  Rate Transition : RateTransition  OutPortSampleTime=0.04
  Scope{1..9} (9 alike) : Scope
      Scope1 settings: ActiveDisplayYMinimum=-1  ActiveDisplayYMaximum=1  DataLoggingVariableName=ScopeData8
      Scope2 settings: ActiveDisplayYMinimum=-0.77251868208460861  ActiveDisplayYMaximum=0.080039739519414982  DataLoggingVariableName=ScopeData7
      Scope3 settings: ActiveDisplayYMinimum=-1  ActiveDisplayYMaximum=1  DataLoggingVariableName=ScopeData8
      Scope4 settings: ActiveDisplayYMinimum=-1  ActiveDisplayYMaximum=1  DataLoggingVariableName=ScopeData9
      Scope5 settings: ActiveDisplayYMinimum=-6.2499999999999982  ActiveDisplayYMaximum=56.25  DataLoggingVariableName=ScopeData10
      Scope6 settings: ActiveDisplayYMinimum=-1.2486948621003993  ActiveDisplayYMaximum=1.2498549846778222  DataLoggingVariableName=ScopeData11
      Scope7 settings: ActiveDisplayYMinimum=-0.87499999999999978  ActiveDisplayYMaximum=7.875  DataLoggingVariableName=ScopeData12
      Scope8 settings: ActiveDisplayYMinimum=-0.91973845897049766  ActiveDisplayYMaximum=8.3026771645702038  DataLoggingVariableName=ScopeData13
      Scope9 settings: ActiveDisplayYMinimum=-9.7701503022243354  ActiveDisplayYMaximum=73.160586445122291  DataLoggingVariableName=ScopeData14
  To Workspace : ToWorkspace  VariableName=controller_reference_log  SampleTime=-1
  Unit Delay : UnitDelay  SampleTime=0.04
  acadosSolve : Subsystem  TreatAsAtomicUnit=on
  parkingLongitudinalController : MATLAB Function  TreatAsAtomicUnit=on
  parkingNMPC : MATLAB Function  TreatAsAtomicUnit=on
  "a_cmd " : Outport
  df_cmd : Outport  Port=2
  dr_cmd : Outport  Port=3
  segment_done : Outport  Port=4
  df_ref_out : Outport  Port=5
  dr_ref_out : Outport  Port=6
  v_ref_out : Outport  Port=7
  a_ref_out : Outport  Port=8
  wires:
  Bus Selector2/5 -> Matrix Concatenate/3, parkingNMPC/5(tdf)  "<front_wheel_angle_rad>"
  parkingNMPC/2(max_q) -> Display1/1
  Bus Selector2/2 -> Matrix Concatenate/2, parkingLongitudinalController/2(ty), parkingNMPC/2(ty)  "<y>"
  Bus Selector2/4 -> parkingNMPC/4(tqw)  "<qw>"
  Bus Selector2/3 -> parkingNMPC/3(tqz)  "<qz>"
  Bus Selector2/1 -> parkingNMPC/1(tx), parkingLongitudinalController/1(tx), Matrix Concatenate/1  "<x>"
  parkingNMPC/1(path_length) -> Display/1
  Bus Selector2/6 -> Matrix Concatenate/4, parkingNMPC/6(tdr)  "<rear_wheel_angle_rad>"
  planning/scenario_planning/scenario_selector/trajectory/1 -> Bus Selector2/1
  X/1 -> parkingNMPC/9(X)
  Y/1 -> parkingNMPC/10(Y)
  parkingNMPC/3(s_now) -> parkingLongitudinalController/5(s_now)
  parkingNMPC/4(ey_now) -> Scope1/1
  qz/1 -> parkingNMPC/11(qz)
  qw/1 -> parkingNMPC/12(qw)
  vx/1 -> parkingNMPC/13(vx), parkingLongitudinalController/6(vx)
  df/1 -> parkingNMPC/15(df)
  dr/1 -> parkingNMPC/16(dr)
  parkingNMPC/5(x_now) -> Display2/1  "x_now"
  From Workspace2/1 -> parkingNMPC/17(veh)
  parkingNMPC/6(longitudinal_mode) -> parkingLongitudinalController/7(longitudinal_mode)
  parkingNMPC/7(df_rate_cmd) -> df_cmd/1
  parkingNMPC/8(dr_rate_cmd) -> dr_cmd/1
  parkingNMPC/9(nmpc_info) -> Demux/1
  Demux/1 -> Scope2/1
  Demux/2 -> Scope3/1
  Demux/3 -> Scope4/1
  Demux/4 -> Scope5/1
  Demux/5 -> Scope6/1
  Demux/6 -> Scope7/1
  Bus Selector2/7 -> Matrix Concatenate/5, parkingNMPC/7(tvx), parkingLongitudinalController/3(tvx)  "<longitudinal_velocity_mps>"
  parkingNMPC/10(segment_done) -> segment_done/1
  active_segment/1 -> parkingNMPC/18(active_segment)
  parkingNMPC/11(endpoint_error) -> Demux1/1
  Demux1/1 -> Scope8/1
  Demux1/2 -> Scope9/1
  Bus Selector2/8 -> Matrix Concatenate/6, parkingLongitudinalController/4(tax), parkingNMPC/8(tax)  "<acceleration_mps2>"
  ax_meas/1 -> parkingNMPC/14(ax_meas)
  MATLAB Function/1(a_cmd_history) -> Rate Transition/1
  parkingLongitudinalController/2(a_ref_out) -> a_ref_out/1
  [park_costmap] -> parkingNMPC/20(costmap)
  Matrix Concatenate/1 -> To Workspace/1
  parkingNMPC/12(df_ref_out) -> df_ref_out/1
  parkingNMPC/13(dr_ref_out) -> dr_ref_out/1
  parkingLongitudinalController/3(v_ref_out) -> v_ref_out/1
  reference_out/1 -> Bus Selector/1
  Bus Selector/1 -> parkingNMPC/21(t_ref)  "<t_ref>"
  Bus Selector/2 -> parkingNMPC/22(s_ref)  "<s_ref>"
  Bus Selector/3 -> parkingNMPC/23(x_ref)  "<x_ref>"
  Bus Selector/4 -> parkingNMPC/24(y_ref)  "<y_ref>"
  Bus Selector/5 -> parkingNMPC/25(psi_ref)  "<psi_ref>"
  Bus Selector/6 -> parkingNMPC/26(v_ref)  "<v_ref>"
  Bus Selector/7 -> parkingNMPC/27(a_ref)  "<a_ref>"
  Bus Selector/8 -> parkingNMPC/28(df_nom)  "<df_nom>"
  Bus Selector/9 -> parkingNMPC/29(dr_nom)  "<dr_nom>"
  Unit Delay/1 -> MATLAB Function/1(a_cmd_previous)
  Rate Transition/1 -> parkingNMPC/19(a_cmd_history)
  parkingLongitudinalController/1(a_cmd) -> Unit Delay/1, "a_cmd "/1

== system ATOM_parking_chain/Vehicle_Model ==
  command : Inport
  rear_steer_commanf : Inport  Port=2
  From Workspace : FromWorkspace  VariableName=veh
  Vehicle Dynamics : Subsystem
  Vehicle internal state : Subsystem
      settings: PortSchema="{\"entries\":[{\"content\":{\"sides\":[{\"content\":{},\"type\":\"ConnectorPlacement.EquallySpacedRectSide\",\"uuid\":\"4a3566d2-c9ed-40f5-9383-803dea843249\"},{\"content\":{\"connectorIds\":[\"Out1\",\"Out2\"],\"side\":\"RIGHT\"},\"type\":\"ConnectorPlacement.EquallySpacedRectSide\",\"uuid\":\"38e6b545-4a7a-4953-bfc7-602e8f089057\"},{\"content\":{\"side\":\"TOP\"},\"type\":\"ConnectorPlacement.EquallySpacedRectSide\",\"uuid\":\"85394c7e-506c-43bc-a81e-512f61060685\"},{\"content\":{\"connectorIds\":[\"In1\"],\"side\":\"BOTTOM\"},\"type\":\"ConnectorPlacement.EquallySpacedRectSide\",\"uuid\":\"97da4b67-3c43-4e7d-b3d8-7f85e7f15c39\"}]},\"type\":\"ConnectorPlacement.EquallySpacedConnector\",\"uuid\":\"d0ddb274-13a9-46fc-8356-ac8c2bb4db82\"}],\"packageUris\":[\"http://schema.mathworks.com/mf0/Connector/R2020b\"],\"version\":\"1.0\"}"
  localization/acceleration function : MATLAB Function  TreatAsAtomicUnit=on
  localization/kinematic_state function : MATLAB Function  TreatAsAtomicUnit=on
  kinematic : Outport
  steer_front : Outport  Port=2
  steer_rear : Outport  Port=3
  accel : Outport  Port=4
  wires:
  From Workspace/1 -> localization/acceleration function/2(veh), localization/kinematic_state function/2(veh)
  Vehicle Dynamics/1(IntState) -> localization/kinematic_state function/1(state), localization/acceleration function/1(state), Vehicle internal state/1(IntState)
  Vehicle internal state/2(steer_rear) -> steer_rear/1
  command/1 -> Vehicle Dynamics/1(command)
  localization/kinematic_state function/1(kinematic) -> kinematic/1
  Vehicle internal state/1(steer_front) -> steer_front/1
  localization/acceleration function/1(accel) -> accel/1
  rear_steer_commanf/1 -> Vehicle Dynamics/2(rear_steer_command)

== system ATOM_parking_chain/Vehicle_Model1 ==
  command : Inport
  rear_steer_commanf : Inport  Port=2
  From Workspace : FromWorkspace  VariableName=veh
  Vehicle Dynamics : Subsystem
  Vehicle internal state : Subsystem
      settings: PortSchema="{\"entries\":[{\"content\":{\"sides\":[{\"content\":{},\"type\":\"ConnectorPlacement.EquallySpacedRectSide\",\"uuid\":\"4a3566d2-c9ed-40f5-9383-803dea843249\"},{\"content\":{\"connectorIds\":[\"Out1\",\"Out2\"],\"side\":\"RIGHT\"},\"type\":\"ConnectorPlacement.EquallySpacedRectSide\",\"uuid\":\"38e6b545-4a7a-4953-bfc7-602e8f089057\"},{\"content\":{\"side\":\"TOP\"},\"type\":\"ConnectorPlacement.EquallySpacedRectSide\",\"uuid\":\"85394c7e-506c-43bc-a81e-512f61060685\"},{\"content\":{\"connectorIds\":[\"In1\"],\"side\":\"BOTTOM\"},\"type\":\"ConnectorPlacement.EquallySpacedRectSide\",\"uuid\":\"97da4b67-3c43-4e7d-b3d8-7f85e7f15c39\"}]},\"type\":\"ConnectorPlacement.EquallySpacedConnector\",\"uuid\":\"d0ddb274-13a9-46fc-8356-ac8c2bb4db82\"}],\"packageUris\":[\"http://schema.mathworks.com/mf0/Connector/R2020b\"],\"version\":\"1.0\"}"
  localization/acceleration function : MATLAB Function  TreatAsAtomicUnit=on
  localization/kinematic_state function : MATLAB Function  TreatAsAtomicUnit=on
  kinematic : Outport
  steer_front : Outport  Port=2
  steer_rear : Outport  Port=3
  accel : Outport  Port=4
  wires:
  From Workspace/1 -> localization/acceleration function/2(veh), localization/kinematic_state function/2(veh)
  Vehicle Dynamics/1(IntState) -> localization/kinematic_state function/1(state), localization/acceleration function/1(state), Vehicle internal state/1(IntState)
  Vehicle internal state/2(steer_rear) -> steer_rear/1
  command/1 -> Vehicle Dynamics/1(command)
  localization/kinematic_state function/1(kinematic) -> kinematic/1
  Vehicle internal state/1(steer_front) -> steer_front/1
  localization/acceleration function/1(accel) -> accel/1
  rear_steer_commanf/1 -> Vehicle Dynamics/2(rear_steer_command)

== system ATOM_parking_chain/Vehicle_Model2 ==
  command : Inport
  rear_steer_commanf : Inport  Port=2
  From Workspace : FromWorkspace  VariableName=veh
  Vehicle Dynamics : Subsystem
  Vehicle internal state : Subsystem
      settings: PortSchema="{\"entries\":[{\"content\":{\"sides\":[{\"content\":{},\"type\":\"ConnectorPlacement.EquallySpacedRectSide\",\"uuid\":\"4a3566d2-c9ed-40f5-9383-803dea843249\"},{\"content\":{\"connectorIds\":[\"Out1\",\"Out2\"],\"side\":\"RIGHT\"},\"type\":\"ConnectorPlacement.EquallySpacedRectSide\",\"uuid\":\"38e6b545-4a7a-4953-bfc7-602e8f089057\"},{\"content\":{\"side\":\"TOP\"},\"type\":\"ConnectorPlacement.EquallySpacedRectSide\",\"uuid\":\"85394c7e-506c-43bc-a81e-512f61060685\"},{\"content\":{\"connectorIds\":[\"In1\"],\"side\":\"BOTTOM\"},\"type\":\"ConnectorPlacement.EquallySpacedRectSide\",\"uuid\":\"97da4b67-3c43-4e7d-b3d8-7f85e7f15c39\"}]},\"type\":\"ConnectorPlacement.EquallySpacedConnector\",\"uuid\":\"d0ddb274-13a9-46fc-8356-ac8c2bb4db82\"}],\"packageUris\":[\"http://schema.mathworks.com/mf0/Connector/R2020b\"],\"version\":\"1.0\"}"
  localization/acceleration function : MATLAB Function  TreatAsAtomicUnit=on
  localization/kinematic_state function : MATLAB Function  TreatAsAtomicUnit=on
  kinematic : Outport
  steer_front : Outport  Port=2
  steer_rear : Outport  Port=3
  accel : Outport  Port=4
  wires:
  From Workspace/1 -> localization/acceleration function/2(veh), localization/kinematic_state function/2(veh)
  Vehicle Dynamics/1(IntState) -> localization/kinematic_state function/1(state), localization/acceleration function/1(state), Vehicle internal state/1(IntState)
  Vehicle internal state/2(steer_rear) -> steer_rear/1
  command/1 -> Vehicle Dynamics/1(command)
  localization/kinematic_state function/1(kinematic) -> kinematic/1
  Vehicle internal state/1(steer_front) -> steer_front/1
  localization/acceleration function/1(accel) -> accel/1
  rear_steer_commanf/1 -> Vehicle Dynamics/2(rear_steer_command)

== system ATOM_parking_chain/parking_velocity_smoother ==
  trajectory_in : Inport
  MATLAB Function : MATLAB Function  TreatAsAtomicUnit=on
  trajectory_out : Outport
  wires:
  trajectory_in/1 -> MATLAB Function/1(trajectory_in)
  MATLAB Function/1(trajectory_out) -> trajectory_out/1

== system ATOM_parking_chain/parking_velocity_smoother1 ==
  trajectory_in : Inport
  MATLAB Function : MATLAB Function  TreatAsAtomicUnit=on
  trajectory_out : Outport
  wires:
  trajectory_in/1 -> MATLAB Function/1(trajectory_in)
  MATLAB Function/1(trajectory_out) -> trajectory_out/1

== system ATOM_parking_chain/parking_velocity_smoother2 ==
  trajectory_in : Inport
  MATLAB Function : MATLAB Function  TreatAsAtomicUnit=on
  trajectory_out : Outport
  wires:
  trajectory_in/1 -> MATLAB Function/1(trajectory_in)
  MATLAB Function/1(trajectory_out) -> trajectory_out/1

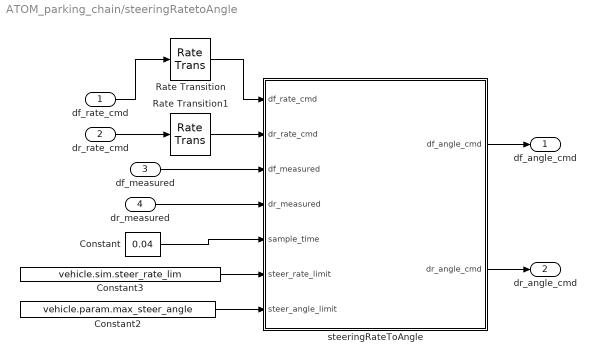
== system ATOM_parking_chain/steeringRatetoAngle ==
  df_rate_cmd : Inport
  dr_rate_cmd : Inport  Port=2
  df_measured : Inport  Port=3
  dr_measured : Inport  Port=4
  Constant : Constant  Value=0.04
  Constant2 : Constant  Value=vehicle.param.max_steer_angle
  Constant3 : Constant  Value=vehicle.sim.steer_rate_lim
  Rate Transition : RateTransition  OutPortSampleTime=0.04
  Rate Transition1 : RateTransition  OutPortSampleTime=0.04
  steeringRateToAngle : MATLAB Function  TreatAsAtomicUnit=on
  df_angle_cmd : Outport
  dr_angle_cmd : Outport  Port=2
  wires:
  steeringRateToAngle/2(dr_angle_cmd) -> dr_angle_cmd/1
  steeringRateToAngle/1(df_angle_cmd) -> df_angle_cmd/1
  dr_measured/1 -> steeringRateToAngle/4(dr_measured)
  df_measured/1 -> steeringRateToAngle/3(df_measured)
  dr_rate_cmd/1 -> Rate Transition1/1
  df_rate_cmd/1 -> Rate Transition/1
  Constant2/1 -> steeringRateToAngle/7(steer_angle_limit)
  Constant3/1 -> steeringRateToAngle/6(steer_rate_limit)
  Constant/1 -> steeringRateToAngle/5(sample_time)
  Rate Transition/1 -> steeringRateToAngle/1(df_rate_cmd)
  Rate Transition1/1 -> steeringRateToAngle/2(dr_rate_cmd)

== system ATOM_parking_chain/steeringRatetoAngle1 ==
  df_rate_cmd : Inport
  dr_rate_cmd : Inport  Port=2
  df_measured : Inport  Port=3
  dr_measured : Inport  Port=4
  Constant : Constant  Value=0.04
  Constant2 : Constant  Value=vehicle.param.max_steer_angle
  Constant3 : Constant  Value=vehicle.sim.steer_rate_lim
  Rate Transition : RateTransition  OutPortSampleTime=0.04
  Rate Transition1 : RateTransition  OutPortSampleTime=0.04
  steeringRateToAngle : MATLAB Function  TreatAsAtomicUnit=on
  df_angle_cmd : Outport
  dr_angle_cmd : Outport  Port=2
  wires:
  steeringRateToAngle/2(dr_angle_cmd) -> dr_angle_cmd/1
  steeringRateToAngle/1(df_angle_cmd) -> df_angle_cmd/1
  dr_measured/1 -> steeringRateToAngle/4(dr_measured)
  df_measured/1 -> steeringRateToAngle/3(df_measured)
  dr_rate_cmd/1 -> Rate Transition1/1
  df_rate_cmd/1 -> Rate Transition/1
  Constant2/1 -> steeringRateToAngle/7(steer_angle_limit)
  Constant3/1 -> steeringRateToAngle/6(steer_rate_limit)
  Constant/1 -> steeringRateToAngle/5(sample_time)
  Rate Transition/1 -> steeringRateToAngle/1(df_rate_cmd)
  Rate Transition1/1 -> steeringRateToAngle/2(dr_rate_cmd)

== system ATOM_parking_chain/steeringRatetoAngle2 ==
  df_rate_cmd : Inport
  dr_rate_cmd : Inport  Port=2
  df_measured : Inport  Port=3
  dr_measured : Inport  Port=4
  Constant : Constant  Value=0.04
  Constant2 : Constant  Value=vehicle.param.max_steer_angle
  Constant3 : Constant  Value=vehicle.sim.steer_rate_lim
  Rate Transition : RateTransition  OutPortSampleTime=0.04
  Rate Transition1 : RateTransition  OutPortSampleTime=0.04
  steeringRateToAngle : MATLAB Function  TreatAsAtomicUnit=on
  df_angle_cmd : Outport
  dr_angle_cmd : Outport  Port=2
  wires:
  steeringRateToAngle/2(dr_angle_cmd) -> dr_angle_cmd/1
  steeringRateToAngle/1(df_angle_cmd) -> df_angle_cmd/1
  dr_measured/1 -> steeringRateToAngle/4(dr_measured)
  df_measured/1 -> steeringRateToAngle/3(df_measured)
  dr_rate_cmd/1 -> Rate Transition1/1
  df_rate_cmd/1 -> Rate Transition/1
  Constant2/1 -> steeringRateToAngle/7(steer_angle_limit)
  Constant3/1 -> steeringRateToAngle/6(steer_rate_limit)
  Constant/1 -> steeringRateToAngle/5(sample_time)
  Rate Transition/1 -> steeringRateToAngle/1(df_rate_cmd)
  Rate Transition1/1 -> steeringRateToAngle/2(dr_rate_cmd)

== system ATOM_parking_chain/time_parameterization ==
  trajectory_in : Inport
  steer_rate_limit : Inport  Port=2
  Time parameterization : MATLAB Function  TreatAsAtomicUnit=on
  reference_out : Outport
  wires:
  trajectory_in/1 -> Time parameterization/1(trajectory_in)
  Time parameterization/1(reference_out) -> reference_out/1
  steer_rate_limit/1 -> Time parameterization/2(steer_rate_limit)

== system ATOM_parking_chain/time_parameterization1 ==
  trajectory_in : Inport
  steer_rate_limit : Inport  Port=2
  Time parameterization : MATLAB Function  TreatAsAtomicUnit=on
  To Workspace : ToWorkspace  VariableName=time_parameterized_reference_log  SaveFormat=Timeseries  SampleTime=-1
  reference_out : Outport
  wires:
  trajectory_in/1 -> Time parameterization/1(trajectory_in)
  Time parameterization/1(reference_out) -> To Workspace/1, reference_out/1
  steer_rate_limit/1 -> Time parameterization/2(steer_rate_limit)
